simulink model "vsi_03a_battery"  (R2026a)
settings: Solver=FixedStepDiscrete  StopTime=Tstop  FixedStep=Ts
PostLoadFcn:
  | run(fullfile(fileparts(get_param('vsi_03a_battery','FileName')), 'params_03a_battery.m'));
InitFcn:
  | run(fullfile(fileparts(get_param('vsi_03a_battery','FileName')), 'params_03a_battery.m'));
values from neighbouring files (symbols this model uses):
  AH_sim = AH_bat*T_h/3600    (= 0.000388888888889)    [params_03a_battery.m]    (also in params_03b_lcl.m = AH_bat)
  P_ch = [-P_bms, 0, P_hold]    [params_03a_battery.m]
  P_dis = [-P_hold, 0, P_bms]    [params_03a_battery.m]
  P_P = P_h    [params_03a_battery.m]    (also in params_03b_lcl.m = [0  0  10e3  10e3])
  Q_Q = Q_h    [params_03a_battery.m]    (also in params_03b_lcl.m = [0  0  -4e3  -4e3])
  R0_bat = Ns*1.5e-3    (= 0.336)    [params_03a_battery.m]
  SOC0 = 0.30    (= 0.3)    [params_03a_battery.m]    (also in params_03b_lcl.m = 0.5)
  SOC_bp = [0    0.05 0.10 0.20 0.30 0.50 0.70 0.80 0.90 0.95 1]    [params_03a_battery.m]
  SOC_ch = [SOC_max - dSOC, SOC_max, SOC_max + 0.02]    [params_03a_battery.m]
  SOC_dis = [SOC_min - 0.02, SOC_min, SOC_min + dSOC]    [params_03a_battery.m]
  t_P = hr(h_P)    [params_03a_battery.m]    (also in params_03b_lcl.m = [0  0.02  0.05  1])
  t_Q = hr(h_Q)    [params_03a_battery.m]    (also in params_03b_lcl.m = [0  0.12  0.12+e  1])
  Vdc = interp1(SOC_bp, V0_bat, SOC0)    [params_03a_battery.m]    (also in params_03b_lcl.m)
undefined symbols (not defined in the file or in its folder): aw_on, b_avg, DiscIntNeverNeededParam, dw_max, I_max, k_delay, Ki_i, Ki_pll, Kp_i, Kp_pll, Kt_i, Lf, Lg, Rf, Rg, t_en, Tc, Ts, Vg_pk, wg
libraries: nesl_utility x11, fl_lib x5, ee_lib x5, eeTransforms x3, batteryecm_lib x1, slpidlib x1, eeGeneralControl x1, eeDiscretePi x1, simulink x1, sl_discontinuities x1
settings Model: Creator=HAKAN SARI  LastModifiedBy=HAKAN SARI
settings SimscapeCC: SimscapeLogType=none

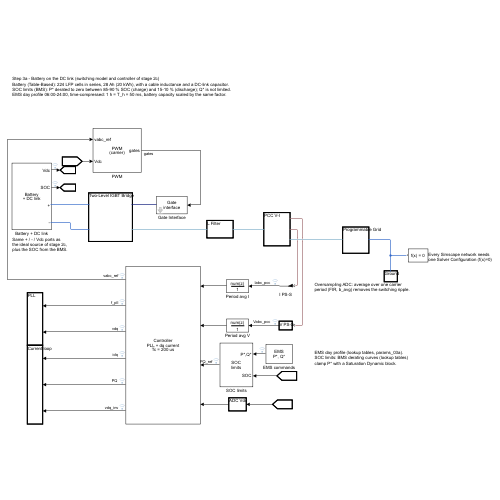
[thumbnail: Simulink's stored preview of the top-level diagram]
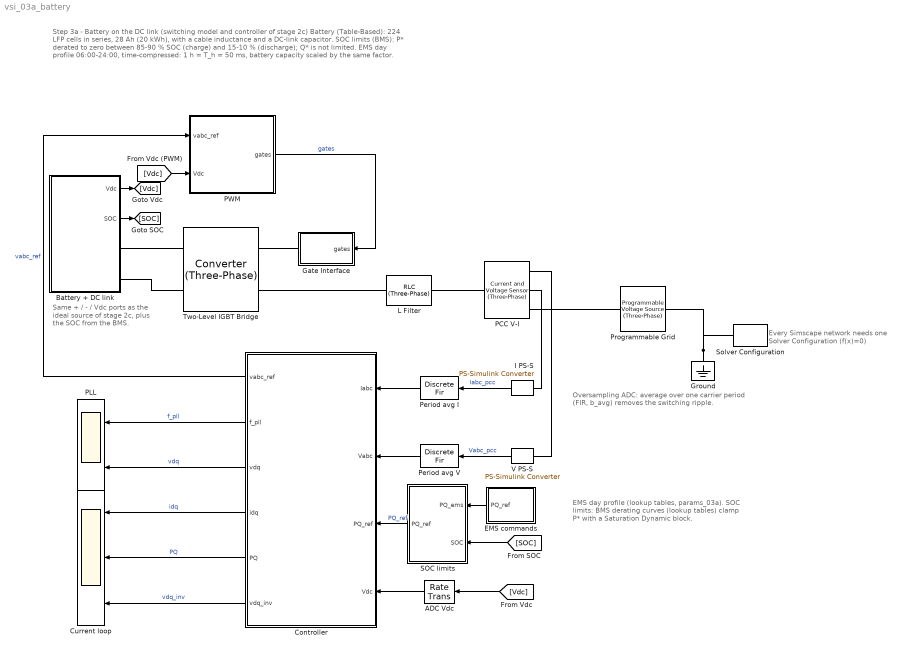
== system vsi_03a_battery ==
  note: Step 3a - Battery on the DC link (switching model and controller of stage 2c)
      | Battery (Table-Based): 224 LFP cells in series, 28 Ah (20 kWh), with a cable inductance and a DC-link capacitor.
      | SOC limits (BMS): P* derated to zero between 85-90 % SOC (charge) and 15-10 % (discharge); Q* is not limited.
      | EMS day profile 06:00-24:00, time-compressed: 1 h = T_h = 50 ms, battery capacity scaled by the same factor.
  note: Every Simscape network needs
      | one Solver Configuration (f(x)=0)
  note: Same + / - / Vdc ports as
      | the ideal source of stage 2c,
      | plus the SOC from the BMS.
  note: Oversampling ADC: average over one carrier
      | period (FIR, b_avg) removes the switching ripple.
  note: EMS day profile (lookup tables, params_03a).
      | SOC limits: BMS derating curves (lookup tables)
      | clamp P* with a Saturation Dynamic block.
  ADC Vdc : RateTransition  OutPortSampleTime=Tc
  Battery + DC link : Subsystem
      mask Display: disp('Battery\n+ DC link');port_label('output',1,'Vdc');port_label('output',2,'SOC');port_label('rconn',1,'+');port_label('rconn',2,'-');
  Controller : Subsystem
      mask Display: disp('Controller\nPLL + dq current\nTc = 200 us');
  Current loop : Scope  NumInputPorts=3
  EMS commands : Subsystem
      mask Display: disp('EMS\nP*, Q*');
  Gate Interface : Subsystem
      mask help: Converts the boolean PWM gate vector [a+ a- b+ b- c+ c-] into the converter gate port (Q1..Q6).
      mask Display: disp('Gate\ninterface');
  Ground : fl_lib/Electrical/Electrical Elements/Electrical Reference
  I PS-S : nesl_utility/PS-Simulink Converter  PhysicalDomain=network_engine_domain  SubClassName=ps_output  LeftPortType=input  RightPortType=output  PseudoPeriodic=off  Frequencies=[]  VectorFormat=1-D array  Unit=inherit  AffineConversion=off
  L Filter : ee_lib/Passive/RLC Assemblies/RLC (Three-Phase)  port_option=ee.enum.threePhasePort.composite  component_structure=4  R=Rf Ohm  L=Lf H  C=1e-6 F  R_parasitic=0 Ohm  G_parasitic=0 1/Ohm  IL_specify=off  IL_priority=High  IL=[0, 0, 0] A  IL_nominal_specify=off  IL_nominal_value=1  IL_nominal_unit=A  VC_specify=off  VC_priority=High  VC=[0, 0, 0] V  VC_nominal_specify=off  VC_nominal_value=1  VC_nominal_unit=V
  PCC V-I : ee_lib/Sensors & Transducers/Current and Voltage Sensor (Three-Phase)  port_option=ee.enum.threePhasePort.composite  vMeasurementType=2  outputUnit=2  SRated=100e6 A*V  VRated=24e3 V  I_specify=off  I_priority=None  I=[0, 0, 0] A  I_nominal_specify=off  I_nominal_value=1  I_nominal_unit=A  V_specify=off  V_priority=None  V=[0, 0, 0] V  V_nominal_specify=off  V_nominal_value=1  V_nominal_unit=V
  PLL : Scope  NumInputPorts=2
  PWM : Subsystem
      mask Display: port_label('input',1,'vabc_ref');port_label('input',2,'Vdc');port_label('output',1,'gates');disp('PWM\n(carrier)');
  Period avg I : DiscreteFir  Coefficients=b_avg  SampleTime=Ts
  Period avg V : DiscreteFir  Coefficients=b_avg  SampleTime=Ts
  Programmable Grid : ee_lib/Sources/Programmable Voltage Source (Three-Phase)  magnitude_type=ee.enum.timechanging.constant  vline_rms=Vg_ll V  magn_ramp=1 V/s  magn_step=1 V  magn_modu_magn=1 V  magn_modu_freq=1 Hz  magn_t1=1 s  magn_t2=2 s  frequency_type=ee.enum.timechanging.constant  freq=fg Hz  freq_ramp=1 Hz/s  freq_step=1 Hz  freq_modu_magn=1 Hz  freq_modu_freq=1 Hz  freq_t1=1 s  freq_t2=2 s  phase_type=ee.enum.timechanging.step  shift=0 deg  phase_ramp=1 deg/s  phase_step=dphi_deg deg  phase_modu_magn=1 deg  phase_modu_freq=1 Hz  phase_t1=t_phase s  phase_t2=inf s  impedance_option=4  SShortCircuit=1e6 A*V  XR=15  R=Rg Ohm  L=Lg H  G_parasitic=1e-6 1/Ohm  harmonic_option=0  harmonic_orders=[5, 7, 11, 13]  harmonic_ratios=[.1, .1, .1, .1]  harmonic_shifts=[0, 0, 0, 0] deg  harmonic_sequences=[1, 1, 1, 1]  harmonic_t1=-inf s  harmonic_t2=inf s  I_specify=off  I_priority=None  I=[0, 0, 0] A  I_nominal_specify=off  I_nominal_value=1  I_nominal_unit=A  V_specify=off  V_priority=None  V=[0, 0, 0] V  V_nominal_specify=off  V_nominal_value=1  V_nominal_unit=V
  SOC limits : Subsystem
      mask Display: disp('SOC\nlimits');port_label('input',1,'P*,Q*');port_label('input',2,'SOC');
  Solver Configuration : nesl_utility/Solver Configuration  PhysicalDomain=network_engine_domain  SubClassName=solver  LeftPortType=input  RightPortType=generic  Tones=[]  Harmonics=[]  SimulateNoise=off  Profile=off  UseLocalSampling=off  EnableSwitchedLinearOptims=on  FrequencyDomain=off  UseCCode=off  RelTol=0.001  AbsTol=0.001  MinStep=1e-09  ToWorkspace=off  RevertToSquareIcSolve=off  NumHomotopyIterations=100  PhasorMode=off  PhasorModeNumHarmonics=1  ConsistencySolver=NEWTON_XTOL_AFTER_FTOL  CanonicalOrdering=CANONICAL  OptimizeIntermediates=OPTIMIZED  IndexReductionMethod=DerivativeReplacement  DoDC=off  ResidualTolerance=1e-09  ConsistencyTolSource=GLOBAL  ConsistencyAbsTol=0.001  ConsistencyRelTol=0.001  ConsistencyTolFactor=0.001  UseLocalSolver=on  LocalSolverChoice=NE_PARTITIONING_ADVANCER  ResolveIndetEquations=on  FunctionEvalNumThread=1  LocalSolverSampleTime=Ts  DoFixedCost=off  MaxNonlinIter=3  MaxModeIter=2  ComputeImpulses=off  ImpulseIterations=2  LinearAlgebra=auto  LinearAlgebraNumThread=0  EquationFormulation=NE_TIME_EF  DelaysMemoryBudget=1024  AutomaticFiltering=on  FilteringTimeConstant=0.001  PartitionStorageMethod=AS_NEEDED  PartitionMemoryBudget=1024  PartitionMethod=ROBUST  MultibodyUseLocalSolver=off  MultibodyLocalSolverChoice=ODE1  MultibodyLocalSolverSampleTime=0.001
  Two-Level IGBT Bridge : ee_lib/Semiconductors & Converters/Converters/Converter (Three-Phase)  port_option=ee.enum.threePhasePort.composite  fidelity_option=ee.enum.converters.fidelity.detailed  device_type=ee.enum.converters.switchingdevice.igbt  showThermalPort=false  K=0  Vth=0.5 V  Vgt=1 V  Vgt_off=-1 V  Ih=1 A  Vf=Vf_sw V  Ron=Ron_sw Ohm  Rds=0.001 Ohm  Goff=1e-6 1/Ohm  Eon_scalar=22.86e-3 J  Eoff_scalar=17.14e-3 J  Eoff_natural_commutation=10e-3 J  Voff=300 V  Iout_scalar=600 A  onCurrentMeasDelay=0 s  useCurrentFromPreviousCycle=false  useVoltageFromPreviousCycle=false  diode_param=ee.enum.converters.protectiondiode.nodynamics  diode_Vf=Vf_sw V  diode_Ron=Ron_sw Ohm  diode_Goff=1e-6 1/Ohm  diode_C=50 nF  diode_iRM=-235 A  diode_iF=300 A  diode_idot=-50 A/us  diode_trr_param=ee.enum.converters.diodetrr.trr_factor  diode_trr_factor=3  diode_trr=15 us  diode_Qrr=1500 s*uA  diode_rec_loss_model=ee.enum.diode.reverseRecoveryModel.fixed  diode_ErecVal=0 J  diode_scaleWithIandV=false  diode_ErecMat=zeros(2, 3) J  diode_TjrecVec=[298.15, 398.15] K  diode_IfrecVec=[.1, 1, 10] A  diode_IrecVal=10 A  diode_VrecVal=10 V  diode_tFilter=1 / 1000 / 100 s  thermal_network_parameterization=ee.enum.thermalNetworkTopology.external  Rth=[.08, .5] K/W  Rth_Cauer=[.08, .1, .5] K/W  Rth_Foster=[.08, .14, .22, .16] K/W  thermal_mass_parameterization=ee.enum.thermalNetwork.timeconstant  thermal_mass=[.01, .5] J/K  thermal_mass_Cauer=[.01, .1, .5] J/K  thermal_mass_Foster=[.001, .005, .05, .5] J/K  thermal_time_constant=[.001, .2] s  thermal_time_constant_Cauer=[.001, .1, .2] s  thermal_time_constant_Foster=[7e-05, .0007, .01, .08] s  thermal_mass_initial_temperatures=[25, 25] degC  thermal_mass_initial_temperatures_Cauer=[25, 25, 25] degC  junction_thermal_mass=0.01 J/K  Tvec_initial_Foster=[25, 25, 25, 25] degC  snubber_type=0  Cs=1e-7 F  Rs=0.1 Ohm  Vce_loss=[0, 150, 300] V
  V PS-S : nesl_utility/PS-Simulink Converter  PhysicalDomain=network_engine_domain  SubClassName=ps_output  LeftPortType=input  RightPortType=output  PseudoPeriodic=off  Frequencies=[]  VectorFormat=1-D array  Unit=inherit  AffineConversion=off
  wires:
  PWM/1(gates) -> Gate Interface/1(gates)  "gates"
  [Vdc] -> PWM/2(Vdc)
  I PS-S/1 -> Period avg I/1  "Iabc_pcc"
  V PS-S/1 -> Period avg V/1  "Vabc_pcc"
  Period avg I/1 -> Controller/1(Iabc)
  Period avg V/1 -> Controller/2(Vabc)
  [Vdc] -> ADC Vdc/1
  ADC Vdc/1 -> Controller/4(Vdc)
  Controller/1(vabc_ref) -> PWM/1(vabc_ref)  "vabc_ref"
  Controller/2(f_pll) -> PLL/1  "f_pll"
  Controller/3(vdq) -> PLL/2  "vdq"
  Controller/4(idq) -> Current loop/1  "idq"
  Controller/5(PQ) -> Current loop/2  "PQ"
  Controller/6(vdq_inv) -> Current loop/3  "vdq_inv"
  Battery + DC link/1(Vdc) -> [Vdc]
  Battery + DC link/2(SOC) -> [SOC]
  EMS commands/1(PQ_ref) -> SOC limits/1(PQ_ems)
  SOC limits/1(PQ_ref) -> Controller/3(PQ_ref)  "PQ_ref"
  [SOC] -> SOC limits/2(SOC)
  connections:
  Two-Level IGBT Bridge/LConn2 -- L Filter/LConn1
  L Filter/RConn1 -- PCC V-I/LConn1
  PCC V-I/RConn3 -- Programmable Grid/RConn1
  Ground/LConn1 -- Programmable Grid/LConn1 -- Solver Configuration/RConn1
  Gate Interface/RConn1 -- Two-Level IGBT Bridge/LConn1
  PCC V-I/RConn2 -- I PS-S/LConn1
  PCC V-I/RConn1 -- V PS-S/LConn1
  Battery + DC link/RConn1 -- Two-Level IGBT Bridge/RConn1
  Battery + DC link/RConn2 -- Two-Level IGBT Bridge/RConn2

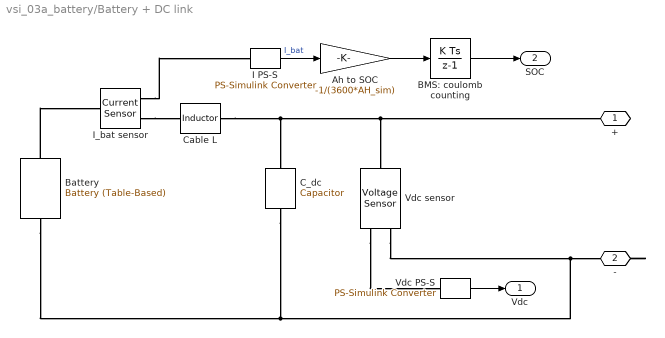
== system vsi_03a_battery/Battery + DC link ==
  Ah to SOC : Gain  Gain=-1/(3600*AH_sim)
  BMS: coulomb counting : DiscreteIntegrator  InitialCondition=SOC0  SampleTime=Ts  ICPrevOutput=DiscIntNeverNeededParam  ICPrevScaledInput=DiscIntNeverNeededParam
  Battery : batteryecm_lib/Battery (Table-Based)  SOC_vec=SOC_bp  T_dependence=simscape.enum.tablebattery.temperature_dependence.no  prm_dir=simscape.enum.tablebattery.prm_dir.noCurrentDirectionality  T_vec=[278, 293, 313] K  V0_mat=[3.49, 3.5, 3.51; 3.55, 3.57, 3.56; 3.62, 3.63, 3.64; 3.71, 3.71, 3.72; 3.91, 3.93, 3.94; 4.07, 4.08, 4.08; 4.19, 4.19, 4.19] V  V0_vec=V0_bat V  V_range=[0, inf] V  R0_mat=[.0117, .0085, .009; .011, .0085, .009; .0114, .0087, .0092; .0107, .0082, .0088; .0107, .0083, .0091; .0113, .0085, .0089; .0116, .0085, .0089] Ohm  R0_vec=R0_bat*ones(size(SOC_bp)) Ohm  R0_dis_mat=[.0117, .0085, .009; .011, .0085, .009; .0114, .0087, .0092; .0107, .0082, .0088; .0107, .0083, .0091; .0113, .0085, .0089; .0116, .0085, .0089] Ohm  R0_dis_vec=[.0085, .0085, .0087, .0082, .0083, .0085, .0085] Ohm  R0_ch_mat=[.0117, .0085, .009; .011, .0085, .009; .0114, .0087, .0092; .0107, .0082, .0088; .0107, .0083, .0091; .0113, .0085, .0089; .0116, .0085, .0089] Ohm  R0_ch_vec=[.0085, .0085, .0087, .0082, .0083, .0085, .0085] Ohm  AH=AH_sim A*hr  prm_leak=simscape.enum.tablebattery.prm_leak.disabled  Rleak_vec=[8000, 7000, 6000] Ohm  Rleak=7e3 Ohm  extrapolation_option=simscape.enum.extrapolation.nearest  SOC_port=simscape.enum.tablebattery.enable.no  prm_dyn=simscape.enum.tablebattery.prm_dyn.off  R1_mat=[.0109, .0029, .0013; .0069, .0024, .0012; .0047, .0026, .0013; .0034, .0016, .001; .0033, .0023, .0014; .0033, .0018, .0011; .0028, .0017, .0011] Ohm  R1_vec=[.0029, .0024, .0026, .0016, .0023, .0018, .0017] Ohm  tau1_mat=[20, 36, 39; 31, 45, 39; 109, 105, 61; 36, 29, 26; 59, 77, 67; 40, 33, 29; 25, 39, 33] s  tau1_vec=[36, 45, 105, 29, 77, 33, 39] s  R2_mat=[.0109, .0029, .0013; .0069, .0024, .0012; .0047, .0026, .0013; .0034, .0016, .001; .0033, .0023, .0014; .0033, .0018, .0011; .0028, .0017, .0011] Ohm  R2_vec=[.0029, .0024, .0026, .0016, .0023, .0018, .0017] Ohm  tau2_mat=[20, 36, 39; 31, 45, 39; 109, 105, 61; 36, 29, 26; 59, 77, 67; 40, 33, 29; 25, 39, 33] s  tau2_vec=[36, 45, 105, 29, 77, 33, 39] s  R3_mat=[.0109, .0029, .0013; .0069, .0024, .0012; .0047, .0026, .0013; .0034, .0016, .001; .0033, .0023, .0014; .0033, .0018, .0011; .0028, .0017, .0011] Ohm  R3_vec=[.0029, .0024, .0026, .0016, .0023, .0018, .0017] Ohm  tau3_mat=[20, 36, 39; 31, 45, 39; 109, 105, 61; 36, 29, 26; 59, 77, 67; 40, 33, 29; 25, 39, 33] s  tau3_vec=[36, 45, 105, 29, 77, 33, 39] s  R4_mat=[.0109, .0029, .0013; .0069, .0024, .0012; .0047, .0026, .0013; .0034, .0016, .001; .0033, .0023, .0014; .0033, .0018, .0011; .0028, .0017, .0011] Ohm  R4_vec=[.0029, .0024, .0026, .0016, .0023, .0018, .0017] Ohm  tau4_mat=[20, 36, 39; 31, 45, 39; 109, 105, 61; 36, 29, 26; 59, 77, 67; 40, 33, 29; 25, 39, 33] s  tau4_vec=[36, 45, 105, 29, 77, 33, 39] s  R5_mat=[.0109, .0029, .0013; .0069, .0024, .0012; .0047, .0026, .0013; .0034, .0016, .001; .0033, .0023, .0014; .0033, .0018, .0011; .0028, .0017, .0011] Ohm  R5_vec=[.0029, .0024, .0026, .0016, .0023, .0018, .0017] Ohm  tau5_mat=[20, 36, 39; 31, 45, 39; 109, 105, 61; 36, 29, 26; 59, 77, 67; 40, 33, 29; 25, 39, 33] s  tau5_vec=[36, 45, 105, 29, 77, 33, 39] s  prm_fade=simscape.enum.tablebattery.prm_fade.disabled  N0=100  dV0=0  dR0=0  dAH=0  dRleak=0  dR1=0  dR2=0  dR3=0  dR4=0  dR5=0  N0vec=[0, 100, 200, 300]  Tfadevec=[298.15, 323.15] K  dV0vec=[0, 0, 0, 0]  dR0vec=[0, 0, 0, 0]  dAHvec=[0, 0, 0, 0]  dRleakvec=[0, 0, 0, 0]  dR1vec=[0, 0, 0, 0]  dR2vec=[0, 0, 0, 0]  dR3vec=[0, 0, 0, 0]  dR4vec=[0, 0, 0, 0]  dR5vec=[0, 0, 0, 0]  dV0mat=[0, 0; 0, 0; 0, 0; 0, 0]  dR0mat=[0, 0; 0, 0; 0, 0; 0, 0]  dAHmat=[0, 0; 0, 0; 0, 0; 0, 0]  dRleakmat=[0, 0; 0, 0; 0, 0; 0, 0]  dR1mat=[0, 0; 0, 0; 0, 0; 0, 0]  dR2mat=[0, 0; 0, 0; 0, 0; 0, 0]  dR3mat=[0, 0; 0, 0; 0, 0; 0, 0]  dR4mat=[0, 0; 0, 0; 0, 0; 0, 0]  dR5mat=[0, 0; 0, 0; 0, 0; 0, 0]  prm_age_modeling=simscape.enum.tablebattery.prm_age_modeling.equation  storage_dt_age_vec=[0] d  storage_T_age_vec=[273] K  prm_age_OCV=simscape.enum.tablebattery.prm_age_OCV.OCV  OCV_age=0.9  SOC_age=0.6  prm_age_resistance=simscape.enum.tablebattery.prm_age.disabled  OCV_scaling_age_resistance=2.2134e6  OCV_offset_age_resistance=1.632e6  temp_exp_age_resistance=0.515833569 V  t_exp_age_resistance=0.75  T_age_vec_resistance=[273.15, 298.15, 323.15] K  dt_age_vec_resistance=[0, 90, 180, 270] d  dR0_age_vec=[0, 0, 0]  t_meas_dR0_age=100 d  dR0_age_mat=[0, 0, 0; 0, 0, 0; 0, 0, 0; 0, 0, 0]  prm_age_capacity=simscape.enum.tablebattery.prm_age.disabled  OCV_scaling_age_capacity=1.5097e07  OCV_offset_age_capacity=8.3625e06  temp_exp_age_capacity=0.6011 V  t_exp_age_capacity=0.75  T_age_vec_capacity=[273.15, 298.15, 323.15] K  dt_age_vec_capacity=[0, 90, 180, 270] d  dAH_age_vec=[0, 0, 0]  t_meas_dAH_age=100 d  dAH_age_mat=[0, 0, 0; 0, 0, 0; 0, 0, 0; 0, 0, 0]  thermal_port=simscape.enum.thermaleffects.omit  temperature=298.15 K  thermal_mass=100 J/K  i_specify=off  i_priority=None  i=0 A  i_nominal_specify=off  i_nominal_value=1  i_nominal_unit=A  v_specify=off  v_priority=None  v=0 V  v_nominal_specify=off  v_nominal_value=1  v_nominal_unit=V  stateOfCharge_specify=on  stateOfCharge_priority=High  stateOfCharge=SOC0  stateOfCharge_nominal_specify=off  stateOfCharge_nominal_value=1  stateOfCharge_nominal_unit=1  num_cycles_specify=off  num_cycles_priority=High  num_cycles=0  num_cycles_nominal_specify=off  num_cycles_nominal_value=1  num_cycles_nominal_unit=1  cell_temperature_specify=off  cell_temperature_priority=High  cell_temperature=298.15 K  cell_temperature_nominal_specify=off  cell_temperature_nominal_value=1  cell_temperature_nominal_unit=K
  C_dc : fl_lib/Electrical/Electrical Elements/Capacitor  c=C_dc F  r=1e-6 Ohm  g=0 1/Ohm  i_specify=off  i_priority=None  i=0 A  i_nominal_specify=off  i_nominal_value=1  i_nominal_unit=A  v_specify=off  v_priority=None  v=0 V  v_nominal_specify=off  v_nominal_value=1  v_nominal_unit=V  vc_specify=on  vc_priority=High  vc=Vdc V  vc_nominal_specify=off  vc_nominal_value=1  vc_nominal_unit=V
  Cable L : fl_lib/Electrical/Electrical Elements/Inductor  l=L_cable H  r=0 Ohm  g=1e-9 1/Ohm  i_specify=off  i_priority=None  i=0 A  i_nominal_specify=off  i_nominal_value=1  i_nominal_unit=A  v_specify=off  v_priority=None  v=0 V  v_nominal_specify=off  v_nominal_value=1  v_nominal_unit=V  i_L_specify=on  i_L_priority=High  i_L=0 A  i_L_nominal_specify=off  i_L_nominal_value=1  i_L_nominal_unit=A
  I PS-S : nesl_utility/PS-Simulink Converter  PhysicalDomain=network_engine_domain  SubClassName=ps_output  LeftPortType=input  RightPortType=output  PseudoPeriodic=off  Frequencies=[]  VectorFormat=inherit  Unit=inherit  AffineConversion=off
  I_bat sensor : fl_lib/Electrical/Electrical Sensors/Current Sensor
  Vdc PS-S : nesl_utility/PS-Simulink Converter  PhysicalDomain=network_engine_domain  SubClassName=ps_output  LeftPortType=input  RightPortType=output  PseudoPeriodic=off  Frequencies=[]  VectorFormat=inherit  Unit=inherit  AffineConversion=off
  Vdc sensor : fl_lib/Electrical/Electrical Sensors/Voltage Sensor
  + : PMIOPort  Side=Right
  - : PMIOPort  Port=2  Side=Right
  Vdc : Outport
  SOC : Outport  Port=2
  wires:
  I PS-S/1 -> Ah to SOC/1  "I_bat"
  Ah to SOC/1 -> BMS: coulomb counting/1
  BMS: coulomb counting/1 -> SOC/1
  Vdc PS-S/1 -> Vdc/1
  connections:
  Battery/LConn1 -- I_bat sensor/LConn1
  I_bat sensor/RConn2 -- Cable L/LConn1
  Cable L/RConn1 -- C_dc/LConn1 -- +/RConn1 -- Vdc sensor/LConn1
  -/RConn1 -- Vdc sensor/RConn2 -- Battery/RConn1 -- C_dc/RConn1
  I_bat sensor/RConn1 -- I PS-S/LConn1
  Vdc sensor/RConn1 -- Vdc PS-S/LConn1

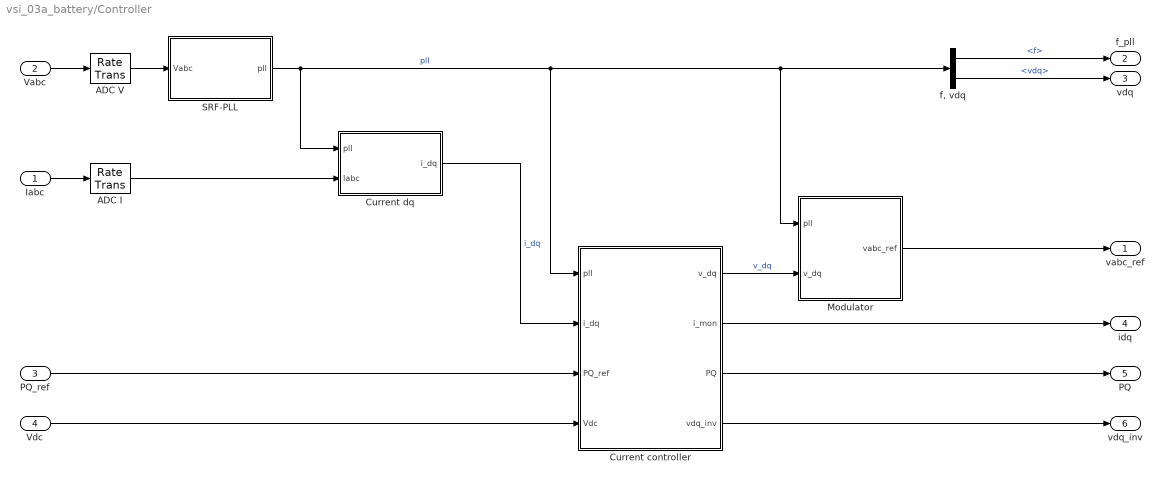
== system vsi_03a_battery/Controller ==
  Iabc : Inport
  Vabc : Inport  Port=2
  PQ_ref : Inport  Port=3
  Vdc : Inport  Port=4
  ADC I : RateTransition  OutPortSampleTime=Tc
  ADC V : RateTransition  OutPortSampleTime=Tc
  Current controller : Subsystem
      mask Display: port_label('input',1,'pll');port_label('input',2,'i_dq');port_label('input',3,'P*,Q*');port_label('input',4,'Vdc');port_label('output',1,'v_dq');port_label('output',2,'i ref/meas');port_label('output',3,'P,Q');port_label('output',4,'v_dq');disp('dq current\ncontroller');
  Current dq : Subsystem
      mask Display: port_label('input',1,'pll');port_label('input',2,'Iabc');disp('abc -> dq');
  Modulator : Subsystem
      mask Display: port_label('input',1,'pll');port_label('input',2,'v_dq');disp('dq -> abc\n+ delay comp.');
  SRF-PLL : Subsystem
      mask Display: disp('SRF-PLL');
  "f, vdq" : BusSelector  OutputSignals=f,vdq
  vabc_ref : Outport
  f_pll : Outport  Port=2
  vdq : Outport  Port=3
  idq : Outport  Port=4
  PQ : Outport  Port=5
  vdq_inv : Outport  Port=6
  wires:
  Current controller/4(vdq_inv) -> vdq_inv/1
  Current controller/3(PQ) -> PQ/1
  Current controller/2(i_mon) -> idq/1
  "f, vdq"/2 -> vdq/1  "<vdq>"
  "f, vdq"/1 -> f_pll/1  "<f>"
  Modulator/1(vabc_ref) -> vabc_ref/1
  Current controller/1(v_dq) -> Modulator/2(v_dq)  "v_dq"
  Vdc/1 -> Current controller/4(Vdc)
  PQ_ref/1 -> Current controller/3(PQ_ref)
  Current dq/1(i_dq) -> Current controller/2(i_dq)  "i_dq"
  SRF-PLL/1(pll) -> Modulator/1(pll), "f, vdq"/1, Current controller/1(pll), Current dq/1(pll)  "pll"
  ADC I/1 -> Current dq/2(Iabc)
  Iabc/1 -> ADC I/1
  ADC V/1 -> SRF-PLL/1(Vabc)
  Vabc/1 -> ADC V/1

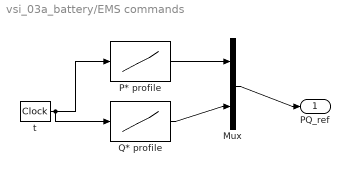
== system vsi_03a_battery/EMS commands ==
  Mux : Mux  Inputs=2
  P* profile : Lookup_n-D  NumberOfTableDimensions=1  BreakpointsForDimension1=t_P  Table=P_P  ExtrapMethod=Clip  InternalRulePriority=Speed  RndMeth=Simplest
  Q* profile : Lookup_n-D  NumberOfTableDimensions=1  BreakpointsForDimension1=t_Q  Table=Q_Q  ExtrapMethod=Clip  InternalRulePriority=Speed  RndMeth=Simplest
  t : DigitalClock  SampleTime=Tc
  PQ_ref : Outport
  wires:
  Mux/1 -> PQ_ref/1
  Q* profile/1 -> Mux/2
  P* profile/1 -> Mux/1
  t/1 -> Q* profile/1, P* profile/1

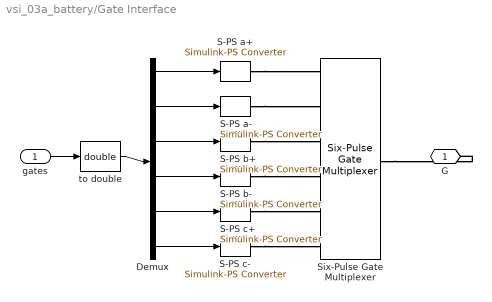
== system vsi_03a_battery/Gate Interface ==
  gates : Inport
  Demux : Demux  Outputs=6
  S-PS a+ : nesl_utility/Simulink-PS Converter  PhysicalDomain=network_engine_domain  SubClassName=ps_input  LeftPortType=input  RightPortType=output  PseudoPeriodic=off  Frequencies=[]  NoiseDistribution=none  NoiseParameters=[]  Unit=1  AffineConversion=off  FilteringAndDerivatives=zero  SimscapeFilterOrder=1  InputFilterTimeConstant=0.001  UdotUserProvided=0
  S-PS a- : nesl_utility/Simulink-PS Converter  PhysicalDomain=network_engine_domain  SubClassName=ps_input  LeftPortType=input  RightPortType=output  PseudoPeriodic=off  Frequencies=[]  NoiseDistribution=none  NoiseParameters=[]  Unit=1  AffineConversion=off  FilteringAndDerivatives=zero  SimscapeFilterOrder=1  InputFilterTimeConstant=0.001  UdotUserProvided=0
  S-PS b+ : nesl_utility/Simulink-PS Converter  PhysicalDomain=network_engine_domain  SubClassName=ps_input  LeftPortType=input  RightPortType=output  PseudoPeriodic=off  Frequencies=[]  NoiseDistribution=none  NoiseParameters=[]  Unit=1  AffineConversion=off  FilteringAndDerivatives=zero  SimscapeFilterOrder=1  InputFilterTimeConstant=0.001  UdotUserProvided=0
  S-PS b- : nesl_utility/Simulink-PS Converter  PhysicalDomain=network_engine_domain  SubClassName=ps_input  LeftPortType=input  RightPortType=output  PseudoPeriodic=off  Frequencies=[]  NoiseDistribution=none  NoiseParameters=[]  Unit=1  AffineConversion=off  FilteringAndDerivatives=zero  SimscapeFilterOrder=1  InputFilterTimeConstant=0.001  UdotUserProvided=0
  S-PS c+ : nesl_utility/Simulink-PS Converter  PhysicalDomain=network_engine_domain  SubClassName=ps_input  LeftPortType=input  RightPortType=output  PseudoPeriodic=off  Frequencies=[]  NoiseDistribution=none  NoiseParameters=[]  Unit=1  AffineConversion=off  FilteringAndDerivatives=zero  SimscapeFilterOrder=1  InputFilterTimeConstant=0.001  UdotUserProvided=0
  S-PS c- : nesl_utility/Simulink-PS Converter  PhysicalDomain=network_engine_domain  SubClassName=ps_input  LeftPortType=input  RightPortType=output  PseudoPeriodic=off  Frequencies=[]  NoiseDistribution=none  NoiseParameters=[]  Unit=1  AffineConversion=off  FilteringAndDerivatives=zero  SimscapeFilterOrder=1  InputFilterTimeConstant=0.001  UdotUserProvided=0
  Six-Pulse Gate Multiplexer : ee_lib/Semiconductors & Converters/Converters/Six-Pulse Gate Multiplexer  port_option=ee.enum.controlport.ps
  to double : DataTypeConversion  OutDataTypeStr=double  SaturateOnIntegerOverflow=off  RndMeth=Floor
  G : PMIOPort  Side=Right
  wires:
  Demux/6 -> S-PS c-/1
  Demux/5 -> S-PS c+/1
  Demux/4 -> S-PS b-/1
  Demux/3 -> S-PS b+/1
  Demux/2 -> S-PS a-/1
  Demux/1 -> S-PS a+/1
  to double/1 -> Demux/1
  gates/1 -> to double/1
  connections:
  Six-Pulse Gate Multiplexer/RConn1 -- G/RConn1
  S-PS c-/RConn1 -- Six-Pulse Gate Multiplexer/LConn6
  S-PS c+/RConn1 -- Six-Pulse Gate Multiplexer/LConn5
  S-PS b-/RConn1 -- Six-Pulse Gate Multiplexer/LConn4
  S-PS b+/RConn1 -- Six-Pulse Gate Multiplexer/LConn3
  S-PS a-/RConn1 -- Six-Pulse Gate Multiplexer/LConn2
  S-PS a+/RConn1 -- Six-Pulse Gate Multiplexer/LConn1

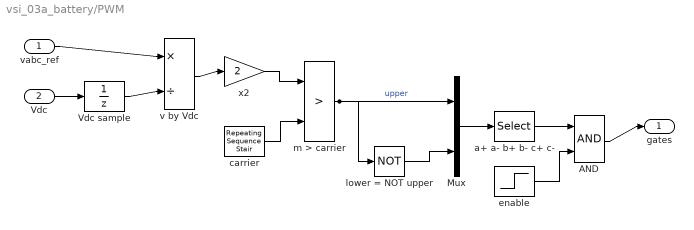
== system vsi_03a_battery/PWM ==
  vabc_ref : Inport
  Vdc : Inport  Port=2
  AND : Logic  AllPortsSameDT=off  OutDataTypeStr=boolean
  Mux : Mux  Inputs=2
  Vdc sample : UnitDelay  InitialCondition=Vdc  SampleTime=Tc
  a+ a- b+ b- c+ c- : Selector  InputPortWidth=6  IndexOptions=Index vector (dialog)  Indices=[1 4 2 5 3 6]  OutputSizes=1
  carrier : simulink/Sources/Repeating Sequence Stair  OutValues=carrier_seq  tsamp=Ts  OutMin=[]  OutMax=[]  OutDataTypeStr=double  OutputDataTypeScalingMode=double  OutDataType=fixdt(0,8)  ConRadixGroup=Best Precision: Vector-wise  OutScaling=2^-12
  enable : Step  Time=t_en  SampleTime=Ts
  lower = NOT upper : Logic  Operator=NOT  AllPortsSameDT=off  OutDataTypeStr=boolean
  m > carrier : RelationalOperator  Operator=>  OutDataTypeStr=boolean  RndMeth=Simplest  InputSameDT=off
  v by Vdc : Product  Inputs=*/
  x2 : Gain  Gain=2
  gates : Outport
  wires:
  vabc_ref/1 -> v by Vdc/1
  Vdc/1 -> Vdc sample/1
  Vdc sample/1 -> v by Vdc/2
  v by Vdc/1 -> x2/1
  x2/1 -> m > carrier/1
  carrier/1 -> m > carrier/2
  m > carrier/1 -> Mux/1, lower = NOT upper/1  "upper"
  lower = NOT upper/1 -> Mux/2
  Mux/1 -> a+ a- b+ b- c+ c-/1
  a+ a- b+ b- c+ c-/1 -> AND/1
  enable/1 -> AND/2
  AND/1 -> gates/1

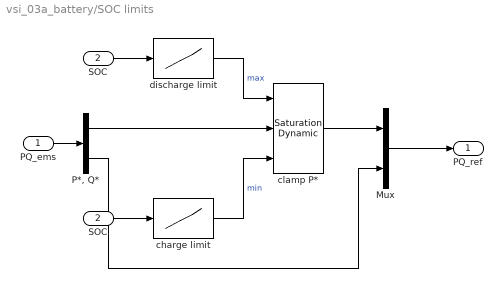
== system vsi_03a_battery/SOC limits ==
  PQ_ems : Inport
  SOC : Inport  Port=2
  Mux : Mux  Inputs=2
  "P*, Q*" : Demux  Outputs=2
  "SOC " : InportShadow  Port=2
  charge limit : Lookup_n-D  NumberOfTableDimensions=1  BreakpointsForDimension1=SOC_ch  Table=P_ch  ExtrapMethod=Clip  InternalRulePriority=Speed  RndMeth=Simplest
  clamp P* : sl_discontinuities/Saturation Dynamic  OutMin=[]  OutMax=[]  OutDataTypeStr=Inherit: Same as second input  OutDataType=fixdt(1, 16)  OutScaling=2^-10  DoSatur=off
      settings: LibrarySourceBlock=|
      | simulink/Discontinuities/Saturation
      | Dynamic
  discharge limit : Lookup_n-D  NumberOfTableDimensions=1  BreakpointsForDimension1=SOC_dis  Table=P_dis  ExtrapMethod=Clip  InternalRulePriority=Speed  RndMeth=Simplest
  PQ_ref : Outport
  wires:
  PQ_ems/1 -> "P*, Q*"/1
  SOC/1 -> discharge limit/1
  "SOC "/1 -> charge limit/1
  "P*, Q*"/1 -> clamp P*/2
  discharge limit/1 -> clamp P*/1  "max"
  charge limit/1 -> clamp P*/3  "min"
  clamp P*/1 -> Mux/1
  "P*, Q*"/2 -> Mux/2
  Mux/1 -> PQ_ref/1

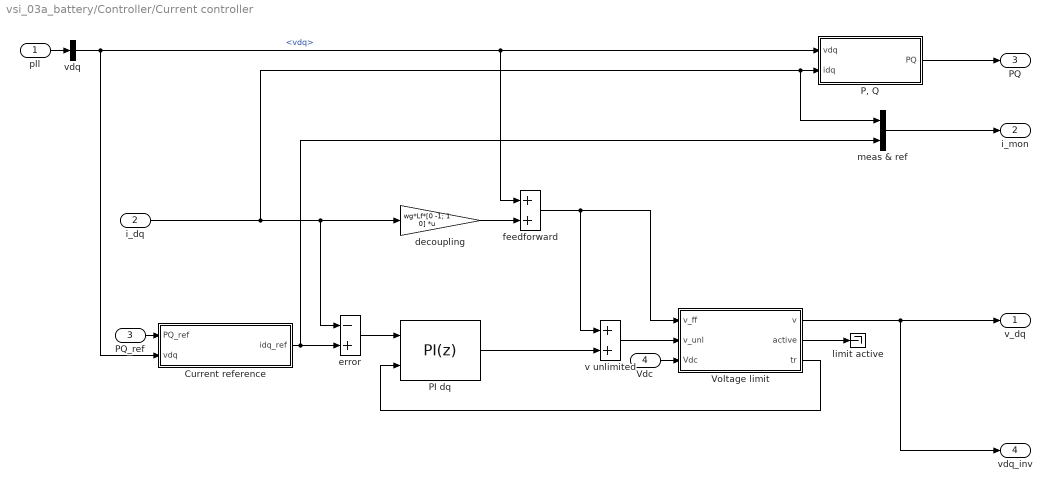
== system vsi_03a_battery/Controller/Current controller ==
  pll : Inport
  i_dq : Inport  Port=2
  PQ_ref : Inport  Port=3
  Vdc : Inport  Port=4
  Current reference : MATLAB Function  TreatAsAtomicUnit=on
  "P, Q" : MATLAB Function  TreatAsAtomicUnit=on
  PI dq : slpidlib/PID Controller  Controller=PI  Form=Parallel  TimeDomain=Discrete-time  UseExternalTs=off  SampleTime=Tc  IntegratorMethod=Forward Euler  FilterMethod=Forward Euler  ControllerParametersSource=internal  P=Kp_i  I=Ki_i  UseKiTs=off  D=0  UseExternalDerivativeSource=off  N=100  UseFilter=on  TunerSelectOption=Transfer Function Based (PID Tuner App)  InitialConditionSource=internal  InitialConditionForIntegrator=0  InitialConditionForFilter=0  DifferentiatorICPrevScaledInput=0  ExternalReset=none  TrackingMode=on  Kt=aw_on*Kt_i  LimitOutput=off  SatLimitsSource=internal  UpperSaturationLimit=inf  LowerSaturationLimit=-inf  LinearizeAsGain=off  AntiWindupMode=none  Kb=1  LimitIntegrator=off  UpperIntegratorSaturationLimit=inf  LowerIntegratorSaturationLimit=-inf  POutMin=[]  POutMax=[]  IOutMin=[]  IOutMax=[]  DOutMin=[]  DOutMax=[]  NOutMin=[]  NOutMax=[]  SumOutMin=[]  SumOutMax=[]  SaturationOutMin=[]  SaturationOutMax=[]  PParamMin=[]  PParamMax=[]  IParamMin=[]  IParamMax=[]  DParamMin=[]  DParamMax=[]  NParamMin=[]  NParamMax=[]  KbParamMin=[]  KbParamMax=[]  KtParamMin=[]  KtParamMax=[]  KbOutMin=[]  KbOutMax=[]  KtOutMin=[]  KtOutMax=[]  IntegratorOutMin=[]  IntegratorOutMax=[]  FilterOutMin=[]  FilterOutMax=[]  SumI1OutMin=[]  SumI1OutMax=[]  SumI2OutMin=[]  SumI2OutMax=[]  SumI3OutMin=[]  SumI3OutMax=[]  SumI4OutMin=[]  SumI4OutMax=[]  SumDOutMin=[]  SumDOutMax=[]  DifferentiatorOutMin=[]  DifferentiatorOutMax=[]  FilterDiffOutCoefMin=[]  FilterDiffOutCoefMax=[]  ReciprocalOutMin=[]  ReciprocalOutMax=[]  SumDenOutMin=[]  SumDenOutMax=[]  SumNumOutMin=[]  SumNumOutMax=[]  DivideOutMin=[]  DivideOutMax=[]  UdiffTsProdOutMin=[]  UdiffTsProdOutMax=[]  NTsProdOutMin=[]  NTsProdOutMax=[]  UintegralTsProdOutMin=[]  UintegralTsProdOutMax=[]  UngainTsProdOutMin=[]  UngainTsProdOutMax=[]  ClampingZeroOutDataTypeStr=Inherit: Inherit via back propagation  ClampingZeroOutMin=[]  ClampingZeroOutMax=[]  FilterDenConstantOutDataTypeStr=Inherit: Inherit via back propagation  FilterDenConstantOutMin=[]  FilterDenConstantOutMax=[]  PCopyOutDataTypeStr=Inherit: Inherit via back propagation  PCopyOutMin=[]  PCopyOutMax=[]  NCopyOutDataTypeStr=Inherit: Inherit via back propagation  NCopyOutMin=[]  NCopyOutMax=[]  IntegratorContinuousStateAttributes=''  IntegratorStateMustResolveToSignalObject=off  IntegratorRTWStateStorageClass=Auto  FilterContinuousStateAttributes=''  FilterStateMustResolveToSignalObject=off  FilterRTWStateStorageClass=Auto  ParallelPVariant=InternalParameters  IdealPVariant=Disabled  IVariant=InternalParameters  DVariant=Disabled  IntegratorVariant=Discrete  SatVariant=Disabled  AWVariant=Passthrough  PCopyVariant=Disabled  TRVariant=Enabled  FdbkBlocksVariant=Forward  IdealPFdbkVariant=Disabled  SatFdbkVariant=Disabled  DerivativeFilterVariant=Disabled  NVariant=Disabled  NCopyVariant=Disabled_SignalSpec  FilterICVariant=Disabled  IntegratorICVariant=InternalICs  ExternalResetVariant=Disabled  TRSumVariant=TrackingMode  SumFdbkVariant=Disabled  SumVariant=Sum_PI  TsampFilterVariant=InternalTs  TsampNgainVariant=Passthrough  TsampIntegralVariant=Disabled_SignalSpec  ExternalSaturationOutDataTypeStr=Inherit: Same as second input  DerivativeSourceVariant=Disabled  PreIntVariant=InternalPreInt
      settings: LibrarySourceBlock=simulink/Discrete/Discrete PID Controller
  Voltage limit : MATLAB Function  TreatAsAtomicUnit=on
  decoupling : Gain  Gain=wg*Lf*[0 -1; 1 0]  Multiplication=Matrix(K*u)
  error : Sum  Inputs=-+
  feedforward : Sum
  limit active : Terminator
  meas & ref : Mux  Inputs=2
  v unlimited : Sum
  vdq : BusSelector  OutputSignals=vdq
  v_dq : Outport
  i_mon : Outport  Port=2
  PQ : Outport  Port=3
  vdq_inv : Outport  Port=4
  wires:
  Voltage limit/3(tr) -> PI dq/2
  feedforward/1 -> Voltage limit/1(v_ff), v unlimited/1
  Voltage limit/2(active) -> limit active/1
  meas & ref/1 -> i_mon/1
  Voltage limit/1(v) -> vdq_inv/1, v_dq/1
  Vdc/1 -> Voltage limit/3(Vdc)
  v unlimited/1 -> Voltage limit/2(v_unl)
  PI dq/1 -> v unlimited/2
  error/1 -> PI dq/1
  PQ_ref/1 -> Current reference/1(PQ_ref)
  decoupling/1 -> feedforward/2
  i_dq/1 -> meas & ref/1, "P, Q"/2(idq), error/1, decoupling/1
  "P, Q"/1(PQ) -> PQ/1
  vdq/1 -> feedforward/1, "P, Q"/1(vdq), Current reference/2(vdq)  "<vdq>"
  pll/1 -> vdq/1
  Current reference/1(idq_ref) -> meas & ref/2, error/2

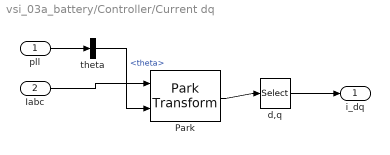
== system vsi_03a_battery/Controller/Current dq ==
  pll : Inport
  Iabc : Inport  Port=2
  Park : eeTransforms/Park Transform  AxisAlignment=Q-axis  PowerInvariant=off
      settings: LibrarySourceBlock=|
      | ee_sl_lib/Mathematical
      | Transforms/Park Transform
  d,q : Selector  InputPortWidth=3  IndexOptions=Index vector (dialog)  Indices=[1 2]  OutputSizes=1
  theta : BusSelector  OutputSignals=theta
  i_dq : Outport
  wires:
  d,q/1 -> i_dq/1
  Park/1 -> d,q/1
  theta/1 -> Park/2  "<theta>"
  Iabc/1 -> Park/1
  pll/1 -> theta/1

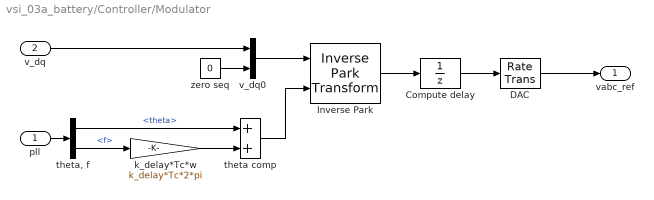
== system vsi_03a_battery/Controller/Modulator ==
  pll : Inport
  v_dq : Inport  Port=2
  Compute delay : UnitDelay  SampleTime=Tc
  DAC : RateTransition  Deterministic=off  OutPortSampleTime=Ts
  Inverse Park : eeTransforms/Inverse Park Transform  AxisAlignment=Q-axis  PowerInvariant=off
      settings: LibrarySourceBlock=|
      | ee_sl_lib/Mathematical
      | Transforms/Inverse
      | Park Transform
  k_delay*Tc*w : Gain  Gain=k_delay*Tc*2*pi
  theta comp : Sum
  "theta, f" : BusSelector  OutputSignals=theta,f
  v_dq0 : Mux  Inputs=2
  zero seq : Constant  Value=0
  vabc_ref : Outport
  wires:
  DAC/1 -> vabc_ref/1
  Compute delay/1 -> DAC/1
  Inverse Park/1 -> Compute delay/1
  theta comp/1 -> Inverse Park/2
  v_dq0/1 -> Inverse Park/1
  zero seq/1 -> v_dq0/2
  v_dq/1 -> v_dq0/1
  k_delay*Tc*w/1 -> theta comp/2
  "theta, f"/2 -> k_delay*Tc*w/1  "<f>"
  "theta, f"/1 -> theta comp/1  "<theta>"
  pll/1 -> "theta, f"/1

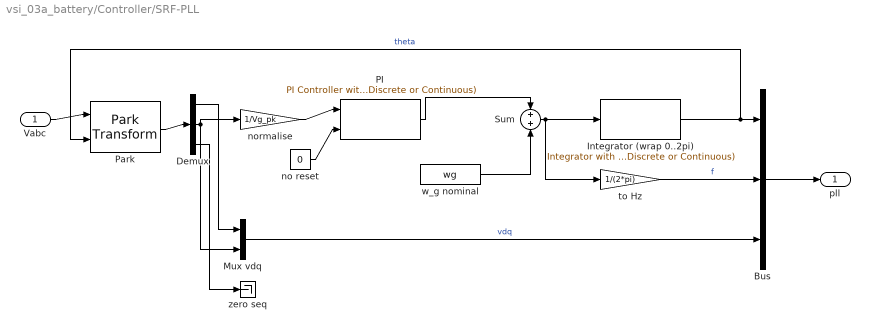
== system vsi_03a_battery/Controller/SRF-PLL ==
  Vabc : Inport
  Bus : BusCreator  Inputs=3
  Demux : Demux  Outputs=3
  Integrator (wrap 0..2pi) : eeGeneralControl/Integrator with Wrapped State (Discrete or Continuous)  LabelModeActiveChoice=Discrete  WrappedStateUpperValue=2*pi  WrappedStateLowerValue=0  x0=0  Ts=Tc
      settings: LibrarySourceBlock=|
      | ee_sl_lib/General Control/Integrator with
      | Wrapped State
      | (Discrete or Continuous)
  Mux vdq : Mux  Inputs=2
  PI : eeDiscretePi/PI Controller with Integral Anti-Windup (Discrete or Continuous)  Kp=Kp_pll  Ki=Ki_pll  x0=0  B=dw_max  A=-dw_max  Ts=Tc
      settings: LibrarySourceBlock=|
      | ee_sl_lib/General Control/PI Controller with
      | Integral Anti-Windup
      | (Discrete or Continuous)
  Park : eeTransforms/Park Transform  AxisAlignment=Q-axis  PowerInvariant=off
      settings: LibrarySourceBlock=|
      | ee_sl_lib/Mathematical
      | Transforms/Park Transform
  Sum : Sum
  no reset : Constant  Value=0  SampleTime=Tc
  normalise : Gain  Gain=1/Vg_pk
  to Hz : Gain  Gain=1/(2*pi)
  w_g nominal : Constant  Value=wg  SampleTime=Tc
  zero seq : Terminator
  pll : Outport
  wires:
  Bus/1 -> pll/1
  Mux vdq/1 -> Bus/3  "vdq"
  Demux/3 -> zero seq/1
  Demux/1 -> Mux vdq/1
  to Hz/1 -> Bus/2  "f"
  Integrator (wrap 0..2pi)/1 -> Park/2, Bus/1  "theta"
  Sum/1 -> to Hz/1, Integrator (wrap 0..2pi)/1
  w_g nominal/1 -> Sum/2
  PI/1 -> Sum/1
  no reset/1 -> PI/2
  normalise/1 -> PI/1
  Demux/2 -> Mux vdq/2, normalise/1
  Park/1 -> Demux/1
  Vabc/1 -> Park/1

== matlab function vsi_03a_battery/Controller/Current controller/Voltage limit ==
  data: v_ff input; v output; v_unl input; Vdc input; active output; tr output
function [v, active, tr] = fcn(v_ff, v_unl, Vdc)
% Linear SPWM: phase peak <= Vdc/2, i.e. |v_dq| <= Vdc/2.
% v_d is mostly the grid-voltage feedforward, v_q is small (~ w*Lf*i_d).
% v_q is kept first and v_d is cut: the d current loop gives way (P drops)
% while the q loop keeps control. Cutting v_q first instead leaves both
% coupled loops without margin and P collapses (try it).
vmax = Vdc/2;
vq = min(max(v_unl(2), -vmax), vmax);
vd_max = sqrt(vmax^2 - vq^2);
vd = min(max(v_unl(1), -vd_max), vd_max);
v = [vd; vq];
active = double(vd ~= v_unl(1) || vq ~= v_unl(2));
% Anti-windup: the PI part that was actually applied. The PI block pulls its
% integrator toward it (tracking input) whenever the limit is active.
tr = v - v_ff;

== matlab function vsi_03a_battery/Controller/Current controller/Current reference ==
  data: PQ_ref input; idq_ref output; vdq input; I_max parameter; Vg_pk parameter
function idq_ref = fcn(PQ_ref, vdq, I_max, Vg_pk)
% i_d* = 2P*/(3 v_d),  i_q* = -2Q*/(3 v_d)   (v_q = 0 when the PLL is locked)
vd = max(vdq(1), 0.5*Vg_pk);              % guard against a collapsed grid voltage
id = 2*PQ_ref(1)/(3*vd);
iq = -2*PQ_ref(2)/(3*vd);
% |i_dq| <= I_max with d-axis (active power) priority
id = min(max(id, -I_max), I_max);
iq_max = sqrt(I_max^2 - id^2);
iq = min(max(iq, -iq_max), iq_max);
idq_ref = [id; iq];

== matlab function vsi_03a_battery/Controller/Current controller/P, Q ==
  data: vdq input; PQ output; idq input
function PQ = fcn(vdq, idq)
% amplitude-invariant dq: P = 1.5(v_d i_d + v_q i_q), Q = 1.5(v_q i_d - v_d i_q)
PQ = 1.5*[vdq(1)*idq(1) + vdq(2)*idq(2); vdq(2)*idq(1) - vdq(1)*idq(2)];
